simulink model "hdlcoder_ofdm_fft_eml"  (R2026a)
settings: Solver=FixedStepDiscrete  StopTime=5000
PreLoadFcn:
  | wordLength = 12;
  | fracLength = 6;
InitFcn:
  | TotalPoint= 512;
  | TotalStage= 9;
  | FFT_nt=numerictype(1,12, 6);
  | twiddle_Signed = 1;
  | twiddle_WordLength = 12;
  | twiddle_FractionLength = 10;
  | twiddle_nt=numerictype(1,12, 10);
undefined symbols (not defined in the file or in its folder): EbNodB, M, Tsym
libraries: hdlsllib x10, commdigbbndam3 x3, dspxfrm3 x2, commsink2 x2, commchan3 x1, simulink x1, commseqgen3 x1, dspindex x1, commrandsrc3 x1
(part 1 of 3)
Description:
  | OFDM Receiver with 512-Point Serial FFT
  | This model shows how to use Simulink(R) HDL Coder(TM) to check, generate,
  | and verify HDL code for a 512-point serial-FFT block built using the
  | MATLAB Function blocks and Simulink(R) blocks.
  | 
  | The 512-point serial-FFT block implements Radix-2 Dicimation-in-Time Cooley-Turkey algorithm.
  | It accepts streaming complex inputs and generate streaming complex outputs.
settings Model: FPTRunName=Active  Creator=The MathWorks, Inc.  LastModifiedBy=The MathWorks, Inc.
settings OptimizationCC: ConditionallyExecuteInputs=off  InitFltsAndDblsToZero=on  EfficientMapNaN2IntZero=off
settings DebuggingCC: AlgebraicLoopMsg=error  MultiTaskDSMMsg=warning  MultiTaskCondExecSysMsg=none  SingleTaskRateTransMsg=error  IntegerOverflowMsg=none  NonBusSignalsTreatedAsBus=error  IntegerSaturationMsg=none
settings HardwareCC: ProdHWDeviceType=32-bit Generic
settings GRTTargetCC: CombineOutputUpdateFcns=off  GRTInterface=on

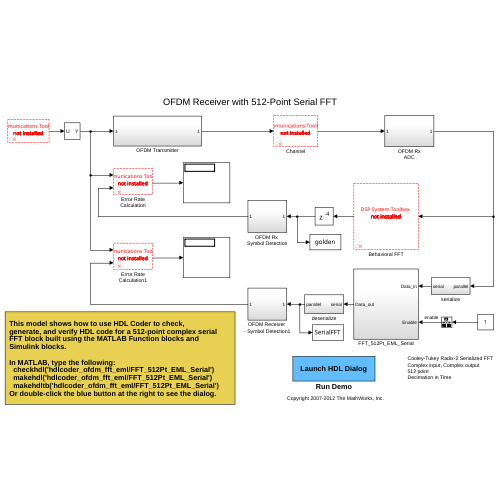
[thumbnail: Simulink's stored preview of the top-level diagram]
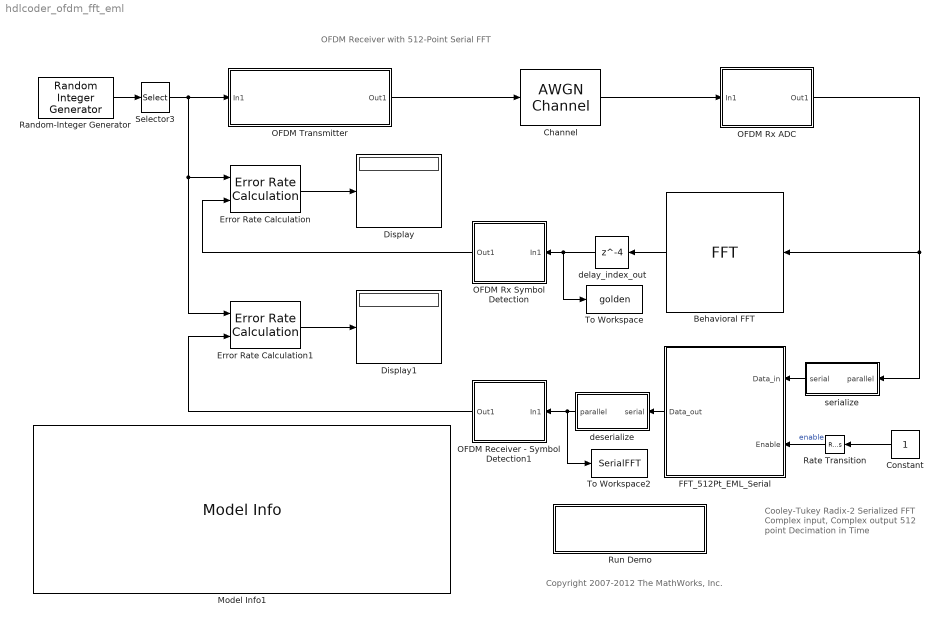
== system hdlcoder_ofdm_fft_eml ==
  note: OFDM Receiver with 512-Point Serial FFT
  note: Cooley-Tukey Radix-2 Serialized FFT
      | Complex input, Complex output
      | 512 point
      | Decimation in Time
  note: Copyright 2007-2012 The MathWorks, Inc.
  Behavioral FFT : dspxfrm3/FFT  FFTImplementation=Auto  CompMethod=Table lookup  TableOpt=NEW  TableOptActive=Speed  BitRevOrder=off  Normalize=off  InheritFFTLength=on  FFTLength=64  WrapInput=on  roundingMode=Floor  overflowMode=off  firstCoeffMode=Specify word length  firstCoeffWordLength=11  firstCoeffFracLength=10  firstCoeffDataTypeStr=fixdt(1,11)  firstCoeffLastDataTypeStr=fixdt(1,11)  prodOutputMode=Binary point scaling  prodOutputWordLength=24  prodOutputFracLength=16  prodOutputDataTypeStr=fixdt(1,24,16)  prodOutputLastDataTypeStr=fixdt(1,24,16)  accumMode=Binary point scaling  accumWordLength=25  accumFracLength=16  accumDataTypeStr=fixdt(1,25,16)  accumLastDataTypeStr=fixdt(1,25,16)  outputMode=Binary point scaling  outputWordLength=12  outputFracLength=6  outputDataTypeStr=fixdt(1,12,6)  outputMin=[]  outputMax=[]  outputLastDataTypeStr=fixdt(1,12,6)
  Channel : commchan3/AWGN Channel  LegacyMode=off  NoiseMethod="Signal to noise ratio  (SNR)"  noiseMode="Signal to noise ratio  (SNR)"  EbNo=10  EsNo=EbNodB+10*log10(log2(M))  SNR=10  BitsPerSymbol=1  SignalPower=1/512  SamplesPerSymbol=round(Tsym / 9.411765e-01)  SymbolPeriod=Tsym  VarianceSource=Parameter  Variance=10^(-0.1*15)/(2048*2)  RandomStream=mt19937ar with seed  Seed=54321  SimulateUsing=Code generation
  Constant : Constant  OutDataTypeStr=boolean  SampleTime=TotalPoint
  Display : Display
  Display1 : Display
  Error Rate Calculation : commsink2/Error Rate Calculation  N=384*4  st_delay=384  cp_mode=Entire frame  subframe=[]  PMode=Port  WsName=ErrorVec  RsMode2=off  stop=off  numErr=100  maxBits=1e6
  Error Rate Calculation1 : commsink2/Error Rate Calculation  N=384*4  st_delay=384  cp_mode=Entire frame  subframe=[]  PMode=Port  WsName=ErrorVec  RsMode2=off  stop=off  numErr=100  maxBits=1e6
  FFT_512Pt_EML_Serial : Subsystem
  Model Info1 : simulink/Model-Wide Utilities/Model Info  Frame=on  DisplayStringWithTags=|  HorizontalTextAlignment=Left  LeftAlignmentValue=0.02
      | This model shows how to use HDL Coder to check, 
      | generate, and verify HDL code for a 512-point complex serial
      | FFT block built using the MATLAB Function blocks and
      | Simulink blocks.
      | 
      | In MATLAB, type the following:
      |   checkhdl('hdlcoder_ofdm_fft_eml/FFT_512Pt_EML_Serial')
      |   makehdl('hdlcoder_ofdm_fft_eml/FFT_512Pt_EML_Serial')
      |   makehdltb('hdlcoder_ofdm_fft_eml/FFT_512Pt_EML_Serial')
      | Or double-click the blue button at the right to see the dialog.
  OFDM Receiver - Symbol Detection1 : Subsystem
  OFDM Rx ADC : Subsystem
  OFDM Rx Symbol Detection : Subsystem
  OFDM Transmitter : Subsystem
  Random-Integer Generator : commrandsrc3/Random Integer Generator  SetSize=64  SeedSource=Parameter  Seed=1234573  SampleTime=1  SamplesPerFrame=512  OutputDataType=uint8  SimulateUsing=Interpreted execution
  Rate Transition : RateTransition
  Run Demo : Subsystem
      settings: OpenFcn=hdldialog(bdroot)
      mask Display: disp('Launch HDL Dialog')
  Selector3 : Selector  InputPortWidth=512  IndexOptions=Index vector (dialog)  Indices=[1:384]  OutputSizes=1
  To Workspace : ToWorkspace  VariableName=golden  SampleTime=-1
      settings: MaxDataPoints=1
  To Workspace2 : ToWorkspace  VariableName=SerialFFT  SampleTime=-1
      settings: MaxDataPoints=1
  delay_index_out : Delay  DelayLength=4  SampleTime=512
  deserialize : Subsystem
  serialize : Subsystem
  wires:
  Channel/1 -> OFDM Rx ADC/1(In1)
  Random-Integer Generator/1 -> Selector3/1
  OFDM Transmitter/1(Out1) -> Channel/1
  Error Rate Calculation1/1 -> Display1/1
  Selector3/1 -> OFDM Transmitter/1(In1), Error Rate Calculation1/1, Error Rate Calculation/1
  FFT_512Pt_EML_Serial/1(Data_out) -> deserialize/1(serial)
  delay_index_out/1 -> OFDM Rx Symbol Detection/1(In1), To Workspace/1
  Behavioral FFT/1 -> delay_index_out/1
  Constant/1 -> Rate Transition/1
  Error Rate Calculation/1 -> Display/1
  serialize/1(serial) -> FFT_512Pt_EML_Serial/1(Data_in)
  Rate Transition/1 -> FFT_512Pt_EML_Serial/2(Enable)  "enable"
  OFDM Rx ADC/1(Out1) -> serialize/1(parallel), Behavioral FFT/1
  deserialize/1(parallel) -> OFDM Receiver - Symbol Detection1/1(In1), To Workspace2/1
  OFDM Rx Symbol Detection/1(Out1) -> Error Rate Calculation/2
  OFDM Receiver - Symbol Detection1/1(Out1) -> Error Rate Calculation1/2

== system hdlcoder_ofdm_fft_eml/FFT_512Pt_EML_Serial ==
  Data_in : Inport
  Enable : Inport  Port=2
  Serialized_FFT : Subsystem
  Terminator : Terminator
  Terminator1 : Terminator
  Data_out : Outport
  wires:
  Enable/1 -> Serialized_FFT/1(enable)
  Data_in/1 -> Serialized_FFT/2(data_in)  "serial_in"
  Serialized_FFT/1(data_en) -> Terminator/1
  Serialized_FFT/2(data_out) -> Data_out/1
  Serialized_FFT/3(Index_out) -> Terminator1/1

== system hdlcoder_ofdm_fft_eml/OFDM Receiver - Symbol Detection1 ==
  In1 : Inport
  Data Type Conversion4 : DataTypeConversion  OutDataTypeStr=uint8  SaturateOnIntegerOverflow=off  RndMeth=Floor
  Extract Data Carriers and Reorder1 : Selector  InputPortWidth=512  IndexOptions=Index vector (dialog)  Indices=[317:340 342:389 391:438 440:487 489:512 2:25 27:74 76:123 125:172 174:197]  OutputSizes=1
  Frame Conversion : FrameConversion
  RX Power Scaling1 : Gain  Gain=1/4
  Rectangular QAM Demodulator Baseband : commdigbbndam3/Rectangular QAM Demodulator Baseband  M=64  OutType=Integer  DecType=Hard decision  VarSource=Dialog  Variance=1  Dec=Gray  Mapping=[0:15]  PowType=Min. distance between symbols  MinDist=2  AvgPow=1  PeakPow=1  Ph=0  outDtype1=Inherit via internal rule  outDtype2=Inherit via internal rule  derotateFactorWordLen=16  derotateFactorDataTypeStr=Inherit: Same word length as input  derotateFactorLastDataTypeStr=Inherit: Same word length as input  denormFactorWordLen=16  denormFactorDataTypeStr=Inherit: Same word length as input  denormFactorLastDataTypeStr=Inherit: Same word length as input  prodOutWordLen=32  prodOutOverflowMode=Wrap  prodOutRoundingMode=Floor  prodOutOvFlMode=off  prodOutOvFlModeLastStrValue=off  sumWordLen=32
  Rx DAC : DataTypeConversion  OutDataTypeStr=double  SaturateOnIntegerOverflow=off  RndMeth=Floor
  Out1 : Outport
  wires:
  In1/1 -> Rx DAC/1
  Data Type Conversion4/1 -> Out1/1
  Extract Data Carriers and Reorder1/1 -> RX Power Scaling1/1
  RX Power Scaling1/1 -> Rectangular QAM Demodulator Baseband/1
  Frame Conversion/1 -> Extract Data Carriers and Reorder1/1
  Rx DAC/1 -> Frame Conversion/1
  Rectangular QAM Demodulator Baseband/1 -> Data Type Conversion4/1

== system hdlcoder_ofdm_fft_eml/OFDM Rx ADC ==
  In1 : Inport
  Frame Conversion1 : FrameConversion  OutFrame=Sample-based
  Remove Cyclic Prefix : Selector  NumberOfDimensions=2  InputPortWidth=80  IndexOptions=Index vector (dialog),Select all  Indices=[33:544],1  OutputSizes=1,1
  Rx ADC : DataTypeConversion  OutDataTypeStr=fixdt(1,wordLength,fracLength)  SaturateOnIntegerOverflow=off  RndMeth=Floor
  Out1 : Outport
  wires:
  Rx ADC/1 -> Frame Conversion1/1
  Frame Conversion1/1 -> Remove Cyclic Prefix/1
  Remove Cyclic Prefix/1 -> Out1/1
  In1/1 -> Rx ADC/1

== system hdlcoder_ofdm_fft_eml/OFDM Rx Symbol Detection ==
  In1 : Inport
  Data Type Conversion4 : DataTypeConversion  OutDataTypeStr=uint8  SaturateOnIntegerOverflow=off  RndMeth=Floor
  Extract Data Carriers and Reorder1 : Selector  InputPortWidth=512  IndexOptions=Index vector (dialog)  Indices=[317:340 342:389 391:438 440:487 489:512 2:25 27:74 76:123 125:172 174:197]  OutputSizes=1
  Frame Conversion : FrameConversion
  RX Power Scaling1 : Gain  Gain=1/4
  Rectangular QAM Demodulator Baseband : commdigbbndam3/Rectangular QAM Demodulator Baseband  M=64  OutType=Integer  DecType=Hard decision  VarSource=Dialog  Variance=1  Dec=Gray  Mapping=[0:15]  PowType=Min. distance between symbols  MinDist=2  AvgPow=1  PeakPow=1  Ph=0  outDtype1=Inherit via internal rule  outDtype2=Inherit via internal rule  derotateFactorWordLen=16  derotateFactorDataTypeStr=Inherit: Same word length as input  derotateFactorLastDataTypeStr=Inherit: Same word length as input  denormFactorWordLen=16  denormFactorDataTypeStr=Inherit: Same word length as input  denormFactorLastDataTypeStr=Inherit: Same word length as input  prodOutWordLen=32  prodOutOverflowMode=Wrap  prodOutRoundingMode=Floor  prodOutOvFlMode=off  prodOutOvFlModeLastStrValue=off  sumWordLen=32
  Rx DAC : DataTypeConversion  OutDataTypeStr=double  SaturateOnIntegerOverflow=off  RndMeth=Floor
  Out1 : Outport
  wires:
  Rectangular QAM Demodulator Baseband/1 -> Data Type Conversion4/1
  Rx DAC/1 -> Frame Conversion/1
  Frame Conversion/1 -> Extract Data Carriers and Reorder1/1
  RX Power Scaling1/1 -> Rectangular QAM Demodulator Baseband/1
  Extract Data Carriers and Reorder1/1 -> RX Power Scaling1/1
  Data Type Conversion4/1 -> Out1/1
  In1/1 -> Rx DAC/1

== system hdlcoder_ofdm_fft_eml/OFDM Transmitter ==
  In1 : Inport
  Append Cyclic Prefix : Selector  NumberOfDimensions=2  InputPortWidth=256  IndexOptions=Index vector (dialog),Select all  Indices=[481:512 1:512],1  OutputSizes=1,1
  IFFT : dspxfrm3/IFFT  FFTImplementation=Auto  CompMethod=Table lookup  TableOpt=HYBRID  TableOptActive=Speed  BitRevOrder=off  cs_in=off  Normalize=on  InheritFFTLength=on  FFTLength=64  WrapInput=on  mode=Complex  outSamplingMode=Frame based  roundingMode=Floor  overflowMode=off  firstCoeffMode=Specify word length  firstCoeffWordLength=16  firstCoeffFracLength=15  firstCoeffDataTypeStr=fixdt(1,16)  firstCoeffLastDataTypeStr=fixdt(1,16)  accumDataTypeStr=Inherit: Same as product output  accumLastDataTypeStr=Inherit: Same as product output  outputMin=[]  outputMax=[]
  Insert Pilots : Subsystem
  Rectangular QAM Modulator Baseband : commdigbbndam3/Rectangular QAM Modulator Baseband  M=64  InType=Integer  Enc=Gray  Mapping=[0:15]  PowType=Min. distance between symbols  MinDist=2  AvgPow=1  PeakPow=1  Ph=0  outDtype=double  outWordLen=16  outUDDataType=sfix(16)  outFracLenMode=Best precision  outFracLen=15  outDataTypeStr=double  outLastDataTypeStr=double
  TX Power Scaling : Gain  Gain=4
  Tx ADC : DataTypeConversion  OutDataTypeStr=fixdt(1,wordLength,fracLength)  SaturateOnIntegerOverflow=off  RndMeth=Floor
  Tx DAC : DataTypeConversion  OutDataTypeStr=double  SaturateOnIntegerOverflow=off  RndMeth=Floor
  Out1 : Outport
  wires:
  Rectangular QAM Modulator Baseband/1 -> Insert Pilots/1(In1)
  Insert Pilots/1(Out1) -> Tx ADC/1
  Tx ADC/1 -> IFFT/1
  TX Power Scaling/1 -> Append Cyclic Prefix/1
  IFFT/1 -> TX Power Scaling/1
  Append Cyclic Prefix/1 -> Tx DAC/1
  In1/1 -> Rectangular QAM Modulator Baseband/1
  Tx DAC/1 -> Out1/1

== system hdlcoder_ofdm_fft_eml/Run Demo ==

== system hdlcoder_ofdm_fft_eml/deserialize ==
  serial : Inport
  Buffer : Buffer  N=512  OutputFrames=off
  Frame Conversion : FrameConversion  OutFrame=Sample-based
  Rate Transition : RateTransition  Deterministic=off  OutPortSampleTime=TotalPoint
  delay_index_out : Delay  DelayLength=238
  tp0c9cbef0_20fa_4817_87de_7b2a1aa0b940 : FrameConversion
  parallel : Outport
  wires:
  delay_index_out/1 -> Buffer/1
  serial/1 -> delay_index_out/1
  Rate Transition/1 -> parallel/1
  Frame Conversion/1 -> Rate Transition/1
  Buffer/1 -> tp0c9cbef0_20fa_4817_87de_7b2a1aa0b940/1
  tp0c9cbef0_20fa_4817_87de_7b2a1aa0b940/1 -> Frame Conversion/1

== system hdlcoder_ofdm_fft_eml/serialize ==
  parallel : Inport
  Frame Conversion : FrameConversion
  Unbuffer : Unbuffer
  serial : Outport
  wires:
  parallel/1 -> Frame Conversion/1
  Frame Conversion/1 -> Unbuffer/1
  Unbuffer/1 -> serial/1

== system hdlcoder_ofdm_fft_eml/FFT_512Pt_EML_Serial/Serialized_FFT ==
  enable : Inport
  data_in : Inport  Port=2
  End_Stage_Reorder : Subsystem
  FFT_Stages : Subsystem
  Start_Stage_BitReverse : Subsystem
  data_en : Outport
  data_out : Outport  Port=2
  Index_out : Outport  Port=3
  wires:
  Start_Stage_BitReverse/1(data_en) -> FFT_Stages/1(enable)
  Start_Stage_BitReverse/2(data_out) -> FFT_Stages/2(data_in)
  enable/1 -> Start_Stage_BitReverse/1(enable)
  data_in/1 -> Start_Stage_BitReverse/2(data_in)
  FFT_Stages/1(data_en) -> End_Stage_Reorder/1(enable)
  FFT_Stages/2(data_out) -> End_Stage_Reorder/2(data_in)
  FFT_Stages/3(index_out) -> End_Stage_Reorder/3(data_in1)
  End_Stage_Reorder/1(data_en) -> data_en/1
  End_Stage_Reorder/2(data_out) -> data_out/1
  End_Stage_Reorder/3(index_out) -> Index_out/1

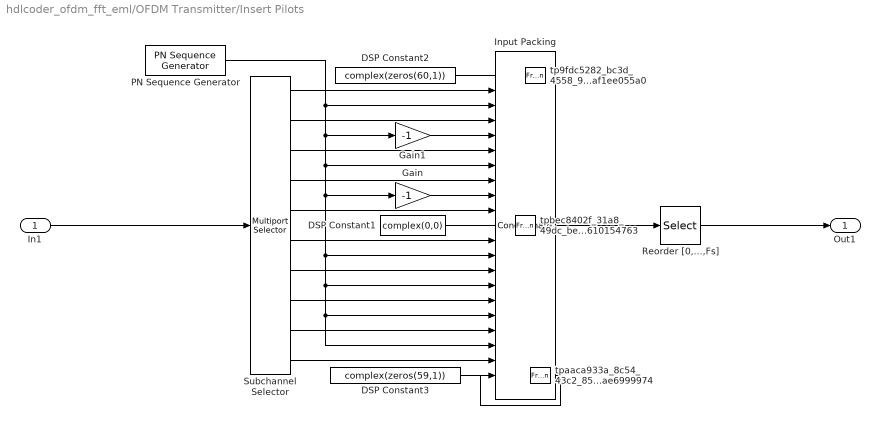
== system hdlcoder_ofdm_fft_eml/OFDM Transmitter/Insert Pilots ==
  In1 : Inport
  DSP Constant1 : Constant  Value=complex(0,0)  VectorParams1D=off
  DSP Constant2 : Constant  Value=complex(zeros(60,1))  VectorParams1D=off
  DSP Constant3 : Constant  Value=complex(zeros(59,1))  VectorParams1D=off
  Gain : Gain  Gain=-1
  Gain1 : Gain  Gain=-1
  Input Packing : Concatenate  NumInputs=21  Mode=Multidimensional array
  PN Sequence Generator : commseqgen3/PN Sequence Generator  poly=[1 0 0 0 0 0 0 0 0 0 0 0 0 1 1]  ini_sta=[1 0 0 1 0 1 0 1 0 0 0 0 0 0]  outBitMaskSource=Dialog parameter  shift=0  outVarSiz=off  maxOutSizeMode=Dialog parameter  maxOutSize=[10 1]  Ts=512  sampPerFrame=1  reset=off  bitPackedOutputs=off  outDataType=double  numPackedBits=8  bitPackDataSigned=off  bitPackedOutDType=double
  Reorder [0,...,Fs] : Selector  NumberOfDimensions=2  InputPortWidth=256  IndexOptions=Index vector (dialog),Select all  Indices=[257:512 1:256],1  OutputSizes=1,1
  Subchannel Selector : dspindex/Multiport Selector  rowsOrCols=Rows  idxCellArray={[1:24],[25:72],[73:120],[121:168],[169:192],[193:216],[217:264],[265:312],[313:360],[361:384]}  idxErrMode=Generate Error
  tp9fdc5282_bc3d_4558_90ac_c7af1ee055a0 : FrameConversion
  tpaaca933a_8c54_43c2_85ab_d0aae6999974 : FrameConversion
  tpbec8402f_31a8_49dc_be14_d26610154763 : FrameConversion
  Out1 : Outport
  wires:
  In1/1 -> Subchannel Selector/1
  PN Sequence Generator/1 -> Gain1/1, Gain/1, Input Packing/19, Input Packing/17, Input Packing/15, Input Packing/13, Input Packing/7, Input Packing/3
  Subchannel Selector/10 -> Input Packing/20
  Subchannel Selector/9 -> Input Packing/18
  Subchannel Selector/8 -> Input Packing/16
  Subchannel Selector/7 -> Input Packing/14
  Subchannel Selector/6 -> Input Packing/12
  Subchannel Selector/5 -> Input Packing/10
  Subchannel Selector/4 -> Input Packing/8
  Subchannel Selector/3 -> Input Packing/6
  Subchannel Selector/2 -> Input Packing/4
  Subchannel Selector/1 -> Input Packing/2
  Gain/1 -> Input Packing/9
  Gain1/1 -> Input Packing/5
  Input Packing/1 -> Reorder [0,...,Fs]/1
  Reorder [0,...,Fs]/1 -> Out1/1
  DSP Constant1/1 -> tpbec8402f_31a8_49dc_be14_d26610154763/1
  tpbec8402f_31a8_49dc_be14_d26610154763/1 -> Input Packing/11
  DSP Constant2/1 -> tp9fdc5282_bc3d_4558_90ac_c7af1ee055a0/1
  tp9fdc5282_bc3d_4558_90ac_c7af1ee055a0/1 -> Input Packing/1
  DSP Constant3/1 -> tpaaca933a_8c54_43c2_85ab_d0aae6999974/1
  tpaaca933a_8c54_43c2_85ab_d0aae6999974/1 -> Input Packing/21

== system hdlcoder_ofdm_fft_eml/FFT_512Pt_EML_Serial/Serialized_FFT/End_Stage_Reorder ==
  enable : Inport
  data_in : Inport  Port=2
  data_in1 : Inport  Port=3
  Data Type Conversion : DataTypeConversion  SaturateOnIntegerOverflow=off  RndMeth=Floor
  Data Type Conversion1 : DataTypeConversion  SaturateOnIntegerOverflow=off  RndMeth=Floor
  Dual Port RAM : hdlsllib/HDL RAMs/Simple Dual Port RAM  ram_size=TotalStage+1
  Reorder_Control_Logics : MATLAB Function  TreatAsAtomicUnit=on
  data_en : Outport
  data_out : Outport  Port=2
  index_out : Outport  Port=3
  wires:
  Data Type Conversion1/1 -> Dual Port RAM/4
  Data Type Conversion/1 -> Dual Port RAM/2
  Reorder_Control_Logics/4(mem_wr_din) -> Dual Port RAM/1
  data_in1/1 -> Reorder_Control_Logics/3(index_in)
  data_in/1 -> Reorder_Control_Logics/2(data_in)
  enable/1 -> Reorder_Control_Logics/1(enable)
  Reorder_Control_Logics/3(index_out) -> index_out/1
  Reorder_Control_Logics/2(data_out) -> data_out/1
  Reorder_Control_Logics/1(data_en) -> data_en/1
  Reorder_Control_Logics/7(mem_rd_addr) -> Data Type Conversion1/1
  Reorder_Control_Logics/6(mem_wr_en) -> Dual Port RAM/3
  Reorder_Control_Logics/5(mem_wr_addr) -> Data Type Conversion/1
  Dual Port RAM/1 -> Reorder_Control_Logics/4(mem_rd_dout)

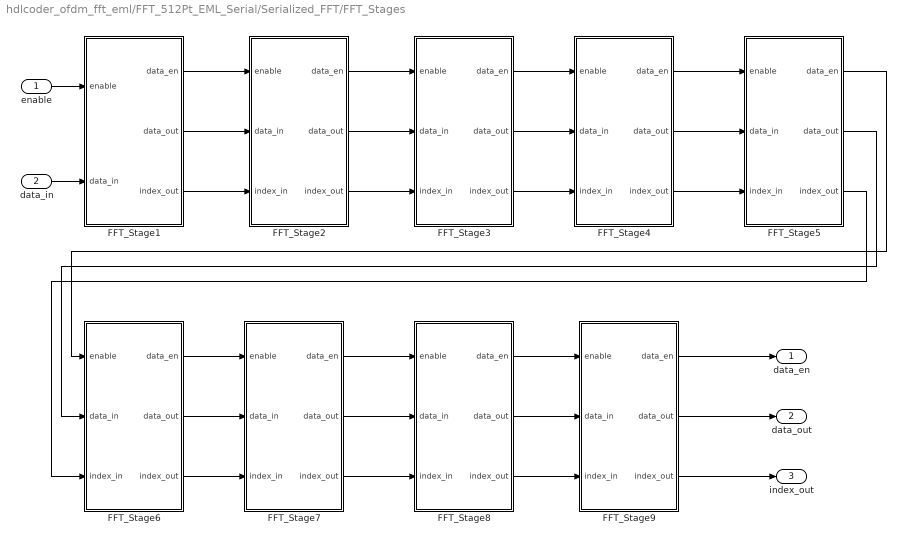
== system hdlcoder_ofdm_fft_eml/FFT_512Pt_EML_Serial/Serialized_FFT/FFT_Stages ==
  enable : Inport
  data_in : Inport  Port=2
  FFT_Stage1 : Subsystem
  FFT_Stage2 : Subsystem
  FFT_Stage3 : Subsystem
  FFT_Stage4 : Subsystem
  FFT_Stage5 : Subsystem
  FFT_Stage6 : Subsystem
  FFT_Stage7 : Subsystem
  FFT_Stage8 : Subsystem
  FFT_Stage9 : Subsystem
  data_en : Outport
  data_out : Outport  Port=2
  index_out : Outport  Port=3
  wires:
  enable/1 -> FFT_Stage1/1(enable)
  data_in/1 -> FFT_Stage1/2(data_in)
  FFT_Stage1/1(data_en) -> FFT_Stage2/1(enable)
  FFT_Stage1/2(data_out) -> FFT_Stage2/2(data_in)
  FFT_Stage1/3(index_out) -> FFT_Stage2/3(index_in)
  FFT_Stage2/1(data_en) -> FFT_Stage3/1(enable)
  FFT_Stage2/2(data_out) -> FFT_Stage3/2(data_in)
  FFT_Stage2/3(index_out) -> FFT_Stage3/3(index_in)
  FFT_Stage3/1(data_en) -> FFT_Stage4/1(enable)
  FFT_Stage3/2(data_out) -> FFT_Stage4/2(data_in)
  FFT_Stage3/3(index_out) -> FFT_Stage4/3(index_in)
  FFT_Stage4/1(data_en) -> FFT_Stage5/1(enable)
  FFT_Stage4/2(data_out) -> FFT_Stage5/2(data_in)
  FFT_Stage4/3(index_out) -> FFT_Stage5/3(index_in)
  FFT_Stage6/1(data_en) -> FFT_Stage7/1(enable)
  FFT_Stage6/2(data_out) -> FFT_Stage7/2(data_in)
  FFT_Stage6/3(index_out) -> FFT_Stage7/3(index_in)
  FFT_Stage7/1(data_en) -> FFT_Stage8/1(enable)
  FFT_Stage7/2(data_out) -> FFT_Stage8/2(data_in)
  FFT_Stage7/3(index_out) -> FFT_Stage8/3(index_in)
  FFT_Stage8/1(data_en) -> FFT_Stage9/1(enable)
  FFT_Stage8/2(data_out) -> FFT_Stage9/2(data_in)
  FFT_Stage8/3(index_out) -> FFT_Stage9/3(index_in)
  FFT_Stage5/1(data_en) -> FFT_Stage6/1(enable)
  FFT_Stage5/2(data_out) -> FFT_Stage6/2(data_in)
  FFT_Stage5/3(index_out) -> FFT_Stage6/3(index_in)
  FFT_Stage9/1(data_en) -> data_en/1
  FFT_Stage9/2(data_out) -> data_out/1
  FFT_Stage9/3(index_out) -> index_out/1

== system hdlcoder_ofdm_fft_eml/FFT_512Pt_EML_Serial/Serialized_FFT/Start_Stage_BitReverse ==
  enable : Inport
  data_in : Inport  Port=2
  BitReverse_Control_Logics : MATLAB Function  TreatAsAtomicUnit=on
  Dual Port RAM : hdlsllib/HDL RAMs/Simple Dual Port RAM  ram_size=TotalStage+1
  delay_data_en : UnitDelay
  delay_data_out : UnitDelay
  data_en : Outport
  data_out : Outport  Port=2
  wires:
  BitReverse_Control_Logics/1(data_en) -> delay_data_en/1
  BitReverse_Control_Logics/2(data_out) -> delay_data_out/1
  enable/1 -> BitReverse_Control_Logics/1(enable)
  data_in/1 -> BitReverse_Control_Logics/2(data_in)
  BitReverse_Control_Logics/3(mem_wr_din) -> Dual Port RAM/1
  BitReverse_Control_Logics/6(mem_rd_addr) -> Dual Port RAM/4
  BitReverse_Control_Logics/5(mem_wr_en) -> Dual Port RAM/3
  BitReverse_Control_Logics/4(mem_wr_addr) -> Dual Port RAM/2
  delay_data_en/1 -> data_en/1
  delay_data_out/1 -> data_out/1
  Dual Port RAM/1 -> BitReverse_Control_Logics/3(mem_rd_dout)

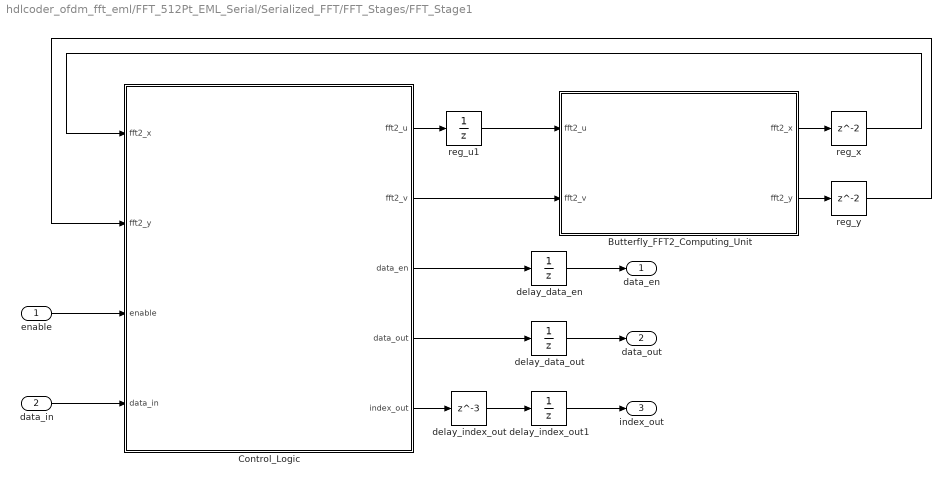
== system hdlcoder_ofdm_fft_eml/FFT_512Pt_EML_Serial/Serialized_FFT/FFT_Stages/FFT_Stage1 ==
  enable : Inport
  data_in : Inport  Port=2
  Butterfly_FFT2_Computing_Unit : MATLAB Function  TreatAsAtomicUnit=on
  Control_Logic : MATLAB Function  TreatAsAtomicUnit=on
  delay_data_en : UnitDelay
  delay_data_out : UnitDelay
  delay_index_out : Delay  DelayLength=3
  delay_index_out1 : UnitDelay
  reg_u1 : UnitDelay
  reg_x : Delay
  reg_y : Delay
  data_en : Outport
  data_out : Outport  Port=2
  index_out : Outport  Port=3
  wires:
  Butterfly_FFT2_Computing_Unit/1(fft2_x) -> reg_x/1
  Butterfly_FFT2_Computing_Unit/2(fft2_y) -> reg_y/1
  delay_index_out/1 -> delay_index_out1/1
  reg_x/1 -> Control_Logic/1(fft2_x)
  reg_y/1 -> Control_Logic/2(fft2_y)
  delay_data_en/1 -> data_en/1
  delay_data_out/1 -> data_out/1
  delay_index_out1/1 -> index_out/1
  Control_Logic/1(fft2_u) -> reg_u1/1
  Control_Logic/2(fft2_v) -> Butterfly_FFT2_Computing_Unit/2(fft2_v)
  reg_u1/1 -> Butterfly_FFT2_Computing_Unit/1(fft2_u)
  enable/1 -> Control_Logic/3(enable)
  data_in/1 -> Control_Logic/4(data_in)
  Control_Logic/3(data_en) -> delay_data_en/1
  Control_Logic/4(data_out) -> delay_data_out/1
  Control_Logic/5(index_out) -> delay_index_out/1

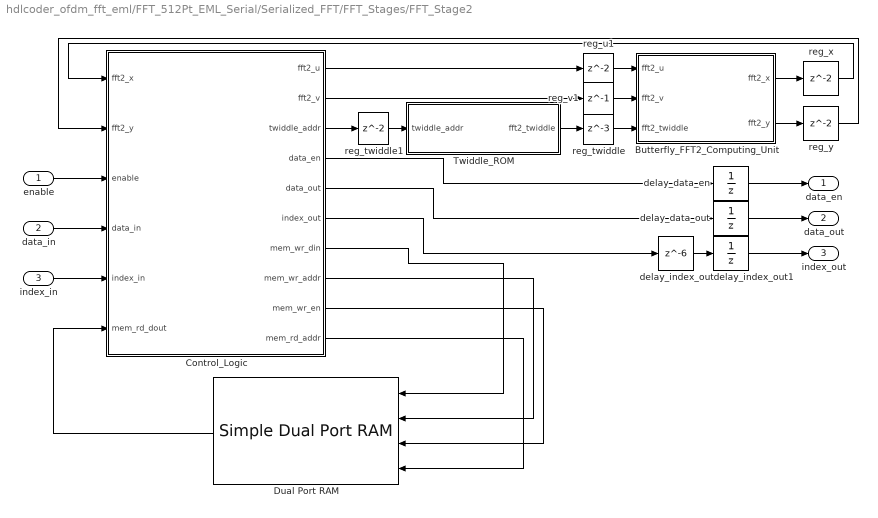
== system hdlcoder_ofdm_fft_eml/FFT_512Pt_EML_Serial/Serialized_FFT/FFT_Stages/FFT_Stage2 ==
  enable : Inport
  data_in : Inport  Port=2
  index_in : Inport  Port=3
  Butterfly_FFT2_Computing_Unit : MATLAB Function  TreatAsAtomicUnit=on
  Control_Logic : MATLAB Function  TreatAsAtomicUnit=on
  Dual Port RAM : hdlsllib/HDL RAMs/Simple Dual Port RAM  ram_size=2
  Twiddle_ROM : MATLAB Function  TreatAsAtomicUnit=on
  delay_data_en : UnitDelay
  delay_data_out : UnitDelay
  delay_index_out : Delay  DelayLength=6
  delay_index_out1 : UnitDelay
  reg_twiddle : Delay  DelayLength=3
  reg_twiddle1 : Delay
  reg_u1 : Delay
  reg_v1 : Delay  DelayLength=1
  reg_x : Delay
  reg_y : Delay
  data_en : Outport
  data_out : Outport  Port=2
  index_out : Outport  Port=3
  wires:
  Control_Logic/7(mem_wr_din) -> Dual Port RAM/1
  Control_Logic/6(index_out) -> delay_index_out/1
  Control_Logic/5(data_out) -> delay_data_out/1
  Control_Logic/4(data_en) -> delay_data_en/1
  Control_Logic/2(fft2_v) -> reg_v1/1
  reg_v1/1 -> Butterfly_FFT2_Computing_Unit/2(fft2_v)
  Dual Port RAM/1 -> Control_Logic/6(mem_rd_dout)
  reg_twiddle1/1 -> Twiddle_ROM/1(twiddle_addr)
  Twiddle_ROM/1(fft2_twiddle) -> reg_twiddle/1
  delay_index_out1/1 -> index_out/1
  delay_data_out/1 -> data_out/1
  delay_data_en/1 -> data_en/1
  index_in/1 -> Control_Logic/5(index_in)
  data_in/1 -> Control_Logic/4(data_in)
  enable/1 -> Control_Logic/3(enable)
  reg_y/1 -> Control_Logic/2(fft2_y)
  reg_x/1 -> Control_Logic/1(fft2_x)
  reg_twiddle/1 -> Butterfly_FFT2_Computing_Unit/3(fft2_twiddle)
  Control_Logic/3(twiddle_addr) -> reg_twiddle1/1
  reg_u1/1 -> Butterfly_FFT2_Computing_Unit/1(fft2_u)
  delay_index_out/1 -> delay_index_out1/1
  Butterfly_FFT2_Computing_Unit/2(fft2_y) -> reg_y/1
  Butterfly_FFT2_Computing_Unit/1(fft2_x) -> reg_x/1
  Control_Logic/1(fft2_u) -> reg_u1/1
  Control_Logic/10(mem_rd_addr) -> Dual Port RAM/4
  Control_Logic/9(mem_wr_en) -> Dual Port RAM/3
  Control_Logic/8(mem_wr_addr) -> Dual Port RAM/2

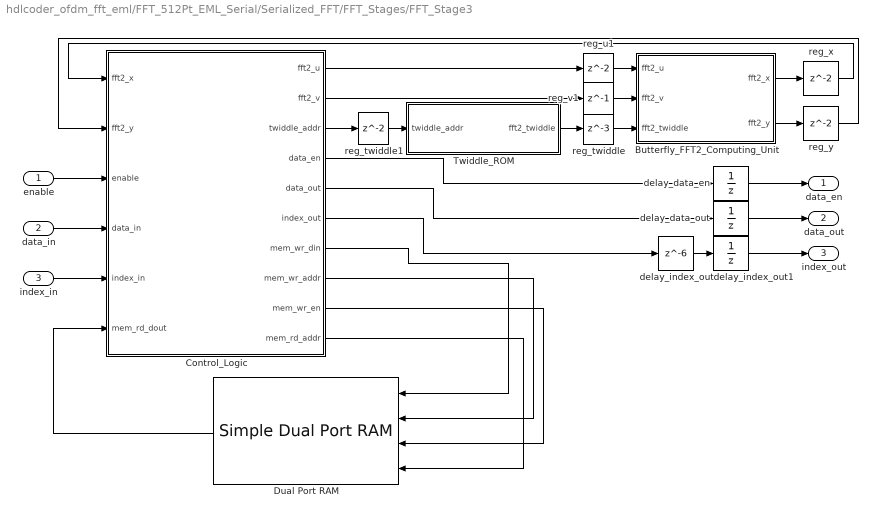
== system hdlcoder_ofdm_fft_eml/FFT_512Pt_EML_Serial/Serialized_FFT/FFT_Stages/FFT_Stage3 ==
  enable : Inport
  data_in : Inport  Port=2
  index_in : Inport  Port=3
  Butterfly_FFT2_Computing_Unit : MATLAB Function  TreatAsAtomicUnit=on
  Control_Logic : MATLAB Function  TreatAsAtomicUnit=on
  Dual Port RAM : hdlsllib/HDL RAMs/Simple Dual Port RAM  ram_size=3
  Twiddle_ROM : MATLAB Function  TreatAsAtomicUnit=on
  delay_data_en : UnitDelay
  delay_data_out : UnitDelay
  delay_index_out : Delay  DelayLength=6
  delay_index_out1 : UnitDelay
  reg_twiddle : Delay  DelayLength=3
  reg_twiddle1 : Delay
  reg_u1 : Delay
  reg_v1 : Delay  DelayLength=1
  reg_x : Delay
  reg_y : Delay
  data_en : Outport
  data_out : Outport  Port=2
  index_out : Outport  Port=3
  wires:
  Control_Logic/8(mem_wr_addr) -> Dual Port RAM/2
  Control_Logic/9(mem_wr_en) -> Dual Port RAM/3
  Control_Logic/10(mem_rd_addr) -> Dual Port RAM/4
  Control_Logic/1(fft2_u) -> reg_u1/1
  Butterfly_FFT2_Computing_Unit/1(fft2_x) -> reg_x/1
  Butterfly_FFT2_Computing_Unit/2(fft2_y) -> reg_y/1
  delay_index_out/1 -> delay_index_out1/1
  reg_u1/1 -> Butterfly_FFT2_Computing_Unit/1(fft2_u)
  Control_Logic/3(twiddle_addr) -> reg_twiddle1/1
  reg_twiddle/1 -> Butterfly_FFT2_Computing_Unit/3(fft2_twiddle)
  reg_x/1 -> Control_Logic/1(fft2_x)
  reg_y/1 -> Control_Logic/2(fft2_y)
  enable/1 -> Control_Logic/3(enable)
  data_in/1 -> Control_Logic/4(data_in)
  index_in/1 -> Control_Logic/5(index_in)
  delay_data_en/1 -> data_en/1
  delay_data_out/1 -> data_out/1
  delay_index_out1/1 -> index_out/1
  Twiddle_ROM/1(fft2_twiddle) -> reg_twiddle/1
  reg_twiddle1/1 -> Twiddle_ROM/1(twiddle_addr)
  Dual Port RAM/1 -> Control_Logic/6(mem_rd_dout)
  reg_v1/1 -> Butterfly_FFT2_Computing_Unit/2(fft2_v)
  Control_Logic/2(fft2_v) -> reg_v1/1
  Control_Logic/4(data_en) -> delay_data_en/1
  Control_Logic/5(data_out) -> delay_data_out/1
  Control_Logic/6(index_out) -> delay_index_out/1
  Control_Logic/7(mem_wr_din) -> Dual Port RAM/1

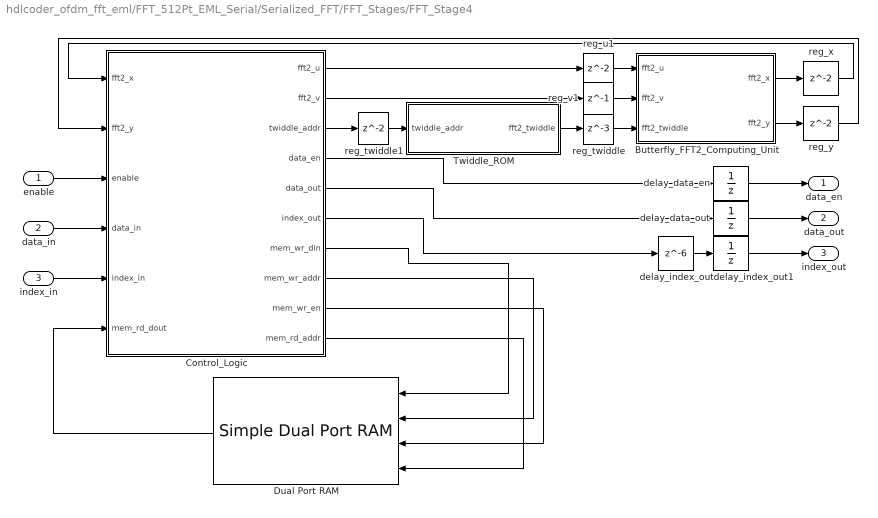
== system hdlcoder_ofdm_fft_eml/FFT_512Pt_EML_Serial/Serialized_FFT/FFT_Stages/FFT_Stage4 ==
  enable : Inport
  data_in : Inport  Port=2
  index_in : Inport  Port=3
  Butterfly_FFT2_Computing_Unit : MATLAB Function  TreatAsAtomicUnit=on
  Control_Logic : MATLAB Function  TreatAsAtomicUnit=on
  Dual Port RAM : hdlsllib/HDL RAMs/Simple Dual Port RAM  ram_size=4
  Twiddle_ROM : MATLAB Function  TreatAsAtomicUnit=on
  delay_data_en : UnitDelay
  delay_data_out : UnitDelay
  delay_index_out : Delay  DelayLength=6
  delay_index_out1 : UnitDelay
  reg_twiddle : Delay  DelayLength=3
  reg_twiddle1 : Delay
  reg_u1 : Delay
  reg_v1 : Delay  DelayLength=1
  reg_x : Delay
  reg_y : Delay
  data_en : Outport
  data_out : Outport  Port=2
  index_out : Outport  Port=3
  wires:
  Control_Logic/7(mem_wr_din) -> Dual Port RAM/1
  Control_Logic/6(index_out) -> delay_index_out/1
  Control_Logic/5(data_out) -> delay_data_out/1
  Control_Logic/4(data_en) -> delay_data_en/1
  Control_Logic/2(fft2_v) -> reg_v1/1
  reg_v1/1 -> Butterfly_FFT2_Computing_Unit/2(fft2_v)
  Dual Port RAM/1 -> Control_Logic/6(mem_rd_dout)
  reg_twiddle1/1 -> Twiddle_ROM/1(twiddle_addr)
  Twiddle_ROM/1(fft2_twiddle) -> reg_twiddle/1
  delay_index_out1/1 -> index_out/1
  delay_data_out/1 -> data_out/1
  delay_data_en/1 -> data_en/1
  index_in/1 -> Control_Logic/5(index_in)
  data_in/1 -> Control_Logic/4(data_in)
  enable/1 -> Control_Logic/3(enable)
  reg_y/1 -> Control_Logic/2(fft2_y)
  reg_x/1 -> Control_Logic/1(fft2_x)
  reg_twiddle/1 -> Butterfly_FFT2_Computing_Unit/3(fft2_twiddle)
  Control_Logic/3(twiddle_addr) -> reg_twiddle1/1
  reg_u1/1 -> Butterfly_FFT2_Computing_Unit/1(fft2_u)
  delay_index_out/1 -> delay_index_out1/1
  Butterfly_FFT2_Computing_Unit/2(fft2_y) -> reg_y/1
  Butterfly_FFT2_Computing_Unit/1(fft2_x) -> reg_x/1
  Control_Logic/1(fft2_u) -> reg_u1/1
  Control_Logic/10(mem_rd_addr) -> Dual Port RAM/4
  Control_Logic/9(mem_wr_en) -> Dual Port RAM/3
  Control_Logic/8(mem_wr_addr) -> Dual Port RAM/2

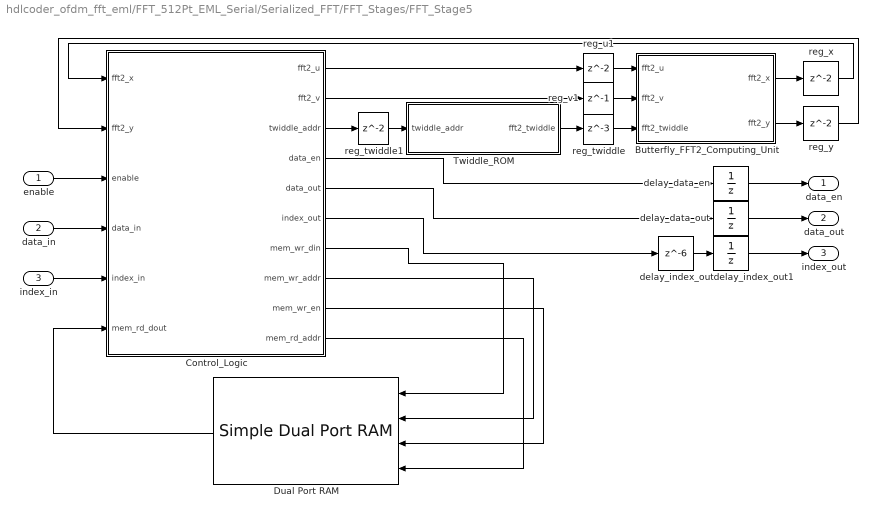
== system hdlcoder_ofdm_fft_eml/FFT_512Pt_EML_Serial/Serialized_FFT/FFT_Stages/FFT_Stage5 ==
  enable : Inport
  data_in : Inport  Port=2
  index_in : Inport  Port=3
  Butterfly_FFT2_Computing_Unit : MATLAB Function  TreatAsAtomicUnit=on
  Control_Logic : MATLAB Function  TreatAsAtomicUnit=on
  Dual Port RAM : hdlsllib/HDL RAMs/Simple Dual Port RAM  ram_size=5
  Twiddle_ROM : MATLAB Function  TreatAsAtomicUnit=on
  delay_data_en : UnitDelay
  delay_data_out : UnitDelay
  delay_index_out : Delay  DelayLength=6
  delay_index_out1 : UnitDelay
  reg_twiddle : Delay  DelayLength=3
  reg_twiddle1 : Delay
  reg_u1 : Delay
  reg_v1 : Delay  DelayLength=1
  reg_x : Delay
  reg_y : Delay
  data_en : Outport
  data_out : Outport  Port=2
  index_out : Outport  Port=3
  wires:
  Control_Logic/8(mem_wr_addr) -> Dual Port RAM/2
  Control_Logic/9(mem_wr_en) -> Dual Port RAM/3
  Control_Logic/10(mem_rd_addr) -> Dual Port RAM/4
  Control_Logic/1(fft2_u) -> reg_u1/1
  Butterfly_FFT2_Computing_Unit/1(fft2_x) -> reg_x/1
  Butterfly_FFT2_Computing_Unit/2(fft2_y) -> reg_y/1
  delay_index_out/1 -> delay_index_out1/1
  reg_u1/1 -> Butterfly_FFT2_Computing_Unit/1(fft2_u)
  Control_Logic/3(twiddle_addr) -> reg_twiddle1/1
  reg_twiddle/1 -> Butterfly_FFT2_Computing_Unit/3(fft2_twiddle)
  reg_x/1 -> Control_Logic/1(fft2_x)
  reg_y/1 -> Control_Logic/2(fft2_y)
  enable/1 -> Control_Logic/3(enable)
  data_in/1 -> Control_Logic/4(data_in)
  index_in/1 -> Control_Logic/5(index_in)
  delay_data_en/1 -> data_en/1
  delay_data_out/1 -> data_out/1
  delay_index_out1/1 -> index_out/1
  Twiddle_ROM/1(fft2_twiddle) -> reg_twiddle/1
  reg_twiddle1/1 -> Twiddle_ROM/1(twiddle_addr)
  Dual Port RAM/1 -> Control_Logic/6(mem_rd_dout)
  reg_v1/1 -> Butterfly_FFT2_Computing_Unit/2(fft2_v)
  Control_Logic/2(fft2_v) -> reg_v1/1
  Control_Logic/4(data_en) -> delay_data_en/1
  Control_Logic/5(data_out) -> delay_data_out/1
  Control_Logic/6(index_out) -> delay_index_out/1
  Control_Logic/7(mem_wr_din) -> Dual Port RAM/1

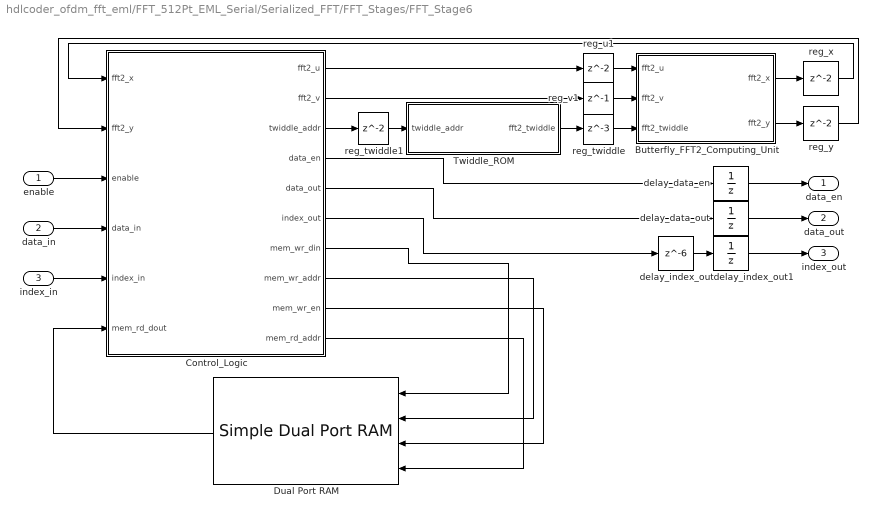
== system hdlcoder_ofdm_fft_eml/FFT_512Pt_EML_Serial/Serialized_FFT/FFT_Stages/FFT_Stage6 ==
  enable : Inport
  data_in : Inport  Port=2
  index_in : Inport  Port=3
  Butterfly_FFT2_Computing_Unit : MATLAB Function  TreatAsAtomicUnit=on
  Control_Logic : MATLAB Function  TreatAsAtomicUnit=on
  Dual Port RAM : hdlsllib/HDL RAMs/Simple Dual Port RAM  ram_size=6
  Twiddle_ROM : MATLAB Function  TreatAsAtomicUnit=on
  delay_data_en : UnitDelay
  delay_data_out : UnitDelay
  delay_index_out : Delay  DelayLength=6
  delay_index_out1 : UnitDelay
  reg_twiddle : Delay  DelayLength=3
  reg_twiddle1 : Delay
  reg_u1 : Delay
  reg_v1 : Delay  DelayLength=1
  reg_x : Delay
  reg_y : Delay
  data_en : Outport
  data_out : Outport  Port=2
  index_out : Outport  Port=3
  wires:
  Control_Logic/7(mem_wr_din) -> Dual Port RAM/1
  Control_Logic/6(index_out) -> delay_index_out/1
  Control_Logic/5(data_out) -> delay_data_out/1
  Control_Logic/4(data_en) -> delay_data_en/1
  Control_Logic/2(fft2_v) -> reg_v1/1
  reg_v1/1 -> Butterfly_FFT2_Computing_Unit/2(fft2_v)
  Dual Port RAM/1 -> Control_Logic/6(mem_rd_dout)
  reg_twiddle1/1 -> Twiddle_ROM/1(twiddle_addr)
  Twiddle_ROM/1(fft2_twiddle) -> reg_twiddle/1
  delay_index_out1/1 -> index_out/1
  delay_data_out/1 -> data_out/1
  delay_data_en/1 -> data_en/1
  index_in/1 -> Control_Logic/5(index_in)
  data_in/1 -> Control_Logic/4(data_in)
  enable/1 -> Control_Logic/3(enable)
  reg_y/1 -> Control_Logic/2(fft2_y)
  reg_x/1 -> Control_Logic/1(fft2_x)
  reg_twiddle/1 -> Butterfly_FFT2_Computing_Unit/3(fft2_twiddle)
  Control_Logic/3(twiddle_addr) -> reg_twiddle1/1
  reg_u1/1 -> Butterfly_FFT2_Computing_Unit/1(fft2_u)
  delay_index_out/1 -> delay_index_out1/1
  Butterfly_FFT2_Computing_Unit/2(fft2_y) -> reg_y/1
  Butterfly_FFT2_Computing_Unit/1(fft2_x) -> reg_x/1
  Control_Logic/1(fft2_u) -> reg_u1/1
  Control_Logic/10(mem_rd_addr) -> Dual Port RAM/4
  Control_Logic/9(mem_wr_en) -> Dual Port RAM/3
  Control_Logic/8(mem_wr_addr) -> Dual Port RAM/2

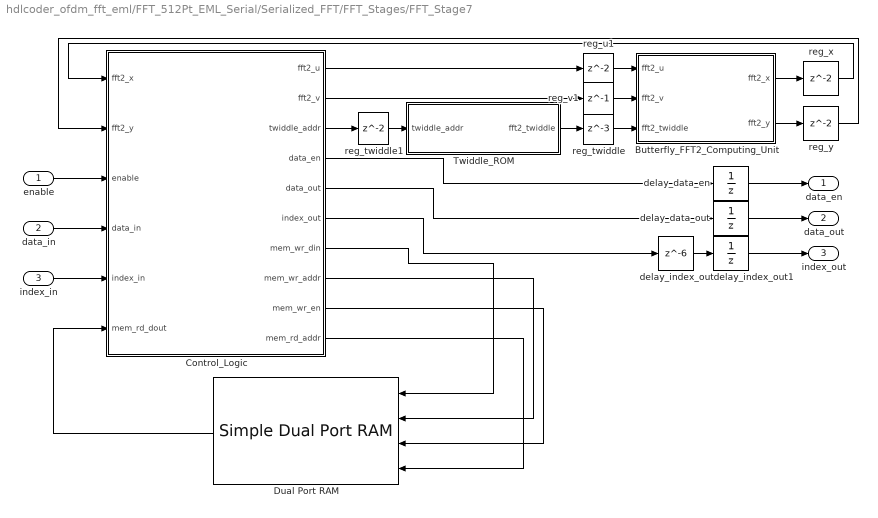
== system hdlcoder_ofdm_fft_eml/FFT_512Pt_EML_Serial/Serialized_FFT/FFT_Stages/FFT_Stage7 ==
  enable : Inport
  data_in : Inport  Port=2
  index_in : Inport  Port=3
  Butterfly_FFT2_Computing_Unit : MATLAB Function  TreatAsAtomicUnit=on
  Control_Logic : MATLAB Function  TreatAsAtomicUnit=on
  Dual Port RAM : hdlsllib/HDL RAMs/Simple Dual Port RAM  ram_size=7
  Twiddle_ROM : MATLAB Function  TreatAsAtomicUnit=on
  delay_data_en : UnitDelay
  delay_data_out : UnitDelay
  delay_index_out : Delay  DelayLength=6
  delay_index_out1 : UnitDelay
  reg_twiddle : Delay  DelayLength=3
  reg_twiddle1 : Delay
  reg_u1 : Delay
  reg_v1 : Delay  DelayLength=1
  reg_x : Delay
  reg_y : Delay
  data_en : Outport
  data_out : Outport  Port=2
  index_out : Outport  Port=3
  wires:
  Control_Logic/8(mem_wr_addr) -> Dual Port RAM/2
  Control_Logic/9(mem_wr_en) -> Dual Port RAM/3
  Control_Logic/10(mem_rd_addr) -> Dual Port RAM/4
  Control_Logic/1(fft2_u) -> reg_u1/1
  Butterfly_FFT2_Computing_Unit/1(fft2_x) -> reg_x/1
  Butterfly_FFT2_Computing_Unit/2(fft2_y) -> reg_y/1
  delay_index_out/1 -> delay_index_out1/1
  reg_u1/1 -> Butterfly_FFT2_Computing_Unit/1(fft2_u)
  Control_Logic/3(twiddle_addr) -> reg_twiddle1/1
  reg_twiddle/1 -> Butterfly_FFT2_Computing_Unit/3(fft2_twiddle)
  reg_x/1 -> Control_Logic/1(fft2_x)
  reg_y/1 -> Control_Logic/2(fft2_y)
  enable/1 -> Control_Logic/3(enable)
  data_in/1 -> Control_Logic/4(data_in)
  index_in/1 -> Control_Logic/5(index_in)
  delay_data_en/1 -> data_en/1
  delay_data_out/1 -> data_out/1
  delay_index_out1/1 -> index_out/1
  Twiddle_ROM/1(fft2_twiddle) -> reg_twiddle/1
  reg_twiddle1/1 -> Twiddle_ROM/1(twiddle_addr)
  Dual Port RAM/1 -> Control_Logic/6(mem_rd_dout)
  reg_v1/1 -> Butterfly_FFT2_Computing_Unit/2(fft2_v)
  Control_Logic/2(fft2_v) -> reg_v1/1
  Control_Logic/4(data_en) -> delay_data_en/1
  Control_Logic/5(data_out) -> delay_data_out/1
  Control_Logic/6(index_out) -> delay_index_out/1
  Control_Logic/7(mem_wr_din) -> Dual Port RAM/1

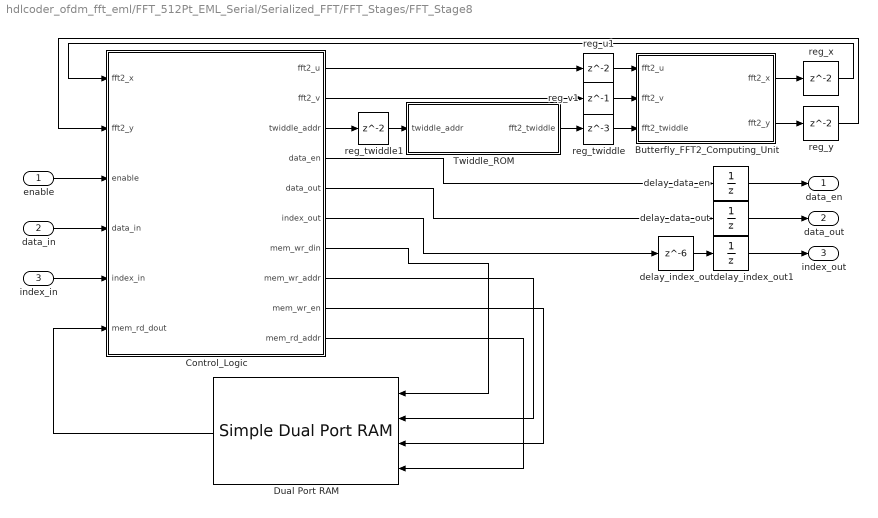
== system hdlcoder_ofdm_fft_eml/FFT_512Pt_EML_Serial/Serialized_FFT/FFT_Stages/FFT_Stage8 ==
  enable : Inport
  data_in : Inport  Port=2
  index_in : Inport  Port=3
  Butterfly_FFT2_Computing_Unit : MATLAB Function  TreatAsAtomicUnit=on
  Control_Logic : MATLAB Function  TreatAsAtomicUnit=on
  Dual Port RAM : hdlsllib/HDL RAMs/Simple Dual Port RAM  ram_size=8
  Twiddle_ROM : MATLAB Function  TreatAsAtomicUnit=on
  delay_data_en : UnitDelay
  delay_data_out : UnitDelay
  delay_index_out : Delay  DelayLength=6
  delay_index_out1 : UnitDelay
  reg_twiddle : Delay  DelayLength=3
  reg_twiddle1 : Delay
  reg_u1 : Delay
  reg_v1 : Delay  DelayLength=1
  reg_x : Delay
  reg_y : Delay
  data_en : Outport
  data_out : Outport  Port=2
  index_out : Outport  Port=3
  wires:
  Control_Logic/7(mem_wr_din) -> Dual Port RAM/1
  Control_Logic/6(index_out) -> delay_index_out/1
  Control_Logic/5(data_out) -> delay_data_out/1
  Control_Logic/4(data_en) -> delay_data_en/1
  Control_Logic/2(fft2_v) -> reg_v1/1
  reg_v1/1 -> Butterfly_FFT2_Computing_Unit/2(fft2_v)
  Dual Port RAM/1 -> Control_Logic/6(mem_rd_dout)
  reg_twiddle1/1 -> Twiddle_ROM/1(twiddle_addr)
  Twiddle_ROM/1(fft2_twiddle) -> reg_twiddle/1
  delay_index_out1/1 -> index_out/1
  delay_data_out/1 -> data_out/1
  delay_data_en/1 -> data_en/1
  index_in/1 -> Control_Logic/5(index_in)
  data_in/1 -> Control_Logic/4(data_in)
  enable/1 -> Control_Logic/3(enable)
  reg_y/1 -> Control_Logic/2(fft2_y)
  reg_x/1 -> Control_Logic/1(fft2_x)
  reg_twiddle/1 -> Butterfly_FFT2_Computing_Unit/3(fft2_twiddle)
  Control_Logic/3(twiddle_addr) -> reg_twiddle1/1
  reg_u1/1 -> Butterfly_FFT2_Computing_Unit/1(fft2_u)
  delay_index_out/1 -> delay_index_out1/1
  Butterfly_FFT2_Computing_Unit/2(fft2_y) -> reg_y/1
  Butterfly_FFT2_Computing_Unit/1(fft2_x) -> reg_x/1
  Control_Logic/1(fft2_u) -> reg_u1/1
  Control_Logic/10(mem_rd_addr) -> Dual Port RAM/4
  Control_Logic/9(mem_wr_en) -> Dual Port RAM/3
  Control_Logic/8(mem_wr_addr) -> Dual Port RAM/2

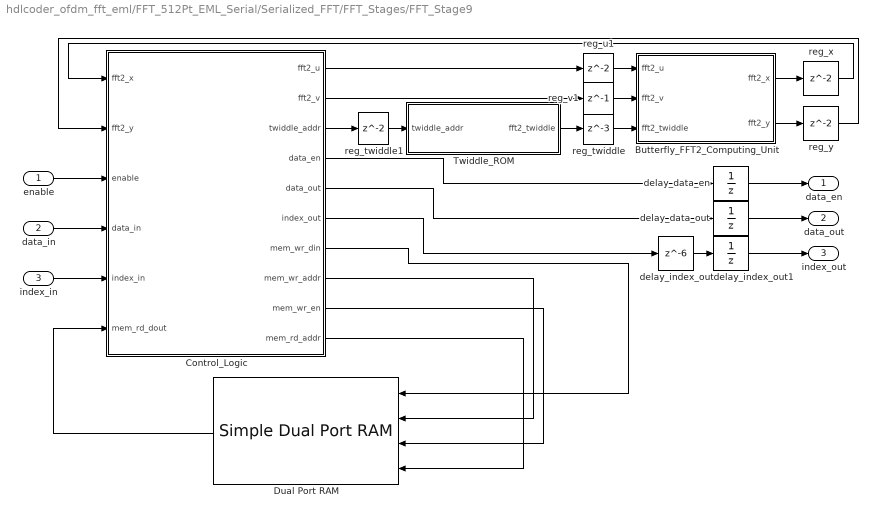
== system hdlcoder_ofdm_fft_eml/FFT_512Pt_EML_Serial/Serialized_FFT/FFT_Stages/FFT_Stage9 ==
  enable : Inport
  data_in : Inport  Port=2
  index_in : Inport  Port=3
  Butterfly_FFT2_Computing_Unit : MATLAB Function  TreatAsAtomicUnit=on
  Control_Logic : MATLAB Function  TreatAsAtomicUnit=on
  Dual Port RAM : hdlsllib/HDL RAMs/Simple Dual Port RAM  ram_size=9
  Twiddle_ROM : MATLAB Function  TreatAsAtomicUnit=on
  delay_data_en : UnitDelay
  delay_data_out : UnitDelay
  delay_index_out : Delay  DelayLength=6
  delay_index_out1 : UnitDelay
  reg_twiddle : Delay  DelayLength=3
  reg_twiddle1 : Delay
  reg_u1 : Delay
  reg_v1 : Delay  DelayLength=1
  reg_x : Delay
  reg_y : Delay
  data_en : Outport
  data_out : Outport  Port=2
  index_out : Outport  Port=3
  wires:
  Control_Logic/7(mem_wr_din) -> Dual Port RAM/1
  Control_Logic/6(index_out) -> delay_index_out/1
  Control_Logic/5(data_out) -> delay_data_out/1
  Control_Logic/4(data_en) -> delay_data_en/1
  Control_Logic/2(fft2_v) -> reg_v1/1
  reg_v1/1 -> Butterfly_FFT2_Computing_Unit/2(fft2_v)
  Dual Port RAM/1 -> Control_Logic/6(mem_rd_dout)
  reg_twiddle1/1 -> Twiddle_ROM/1(twiddle_addr)
  Twiddle_ROM/1(fft2_twiddle) -> reg_twiddle/1
  delay_index_out1/1 -> index_out/1
  delay_data_out/1 -> data_out/1
  delay_data_en/1 -> data_en/1
  index_in/1 -> Control_Logic/5(index_in)
  data_in/1 -> Control_Logic/4(data_in)
  enable/1 -> Control_Logic/3(enable)
  reg_y/1 -> Control_Logic/2(fft2_y)
  reg_x/1 -> Control_Logic/1(fft2_x)
  reg_twiddle/1 -> Butterfly_FFT2_Computing_Unit/3(fft2_twiddle)
  Control_Logic/3(twiddle_addr) -> reg_twiddle1/1
  reg_u1/1 -> Butterfly_FFT2_Computing_Unit/1(fft2_u)
  delay_index_out/1 -> delay_index_out1/1
  Butterfly_FFT2_Computing_Unit/2(fft2_y) -> reg_y/1
  Butterfly_FFT2_Computing_Unit/1(fft2_x) -> reg_x/1
  Control_Logic/1(fft2_u) -> reg_u1/1
  Control_Logic/10(mem_rd_addr) -> Dual Port RAM/4
  Control_Logic/9(mem_wr_en) -> Dual Port RAM/3
  Control_Logic/8(mem_wr_addr) -> Dual Port RAM/2

== matlab function hdlcoder_ofdm_fft_eml/FFT_512Pt_EML_Serial/Serialized_FFT/FFT_Stages/FFT_Stage3/Butterfly_FFT2_Computing_Unit ==
  settings: fimath=hdlfimath
  data: fft2_u input FFT_nt; fft2_x output FFT_nt; fft2_v input FFT_nt; fft2_twiddle input twiddle_nt; fft2_y output FFT_nt
function [fft2_x, fft2_y] = fcn(fft2_u, fft2_v, fft2_twiddle)
% FFT2 Computing Unit

% Scale down number for this stage. Need to be power of 2.
Scale = 1;

% Call function in hdlcoder_serial_fft_butterfly_scale.m on path 
[x, y] = hdlcoder_serial_fft_butterfly(fft2_u, fft2_v, fft2_twiddle);

% scaling down by 2 for each FFT2 stage.
fft2_x = bitsra(x, log2(Scale));
fft2_y = bitsra(y, log2(Scale));

== matlab function hdlcoder_ofdm_fft_eml/FFT_512Pt_EML_Serial/Serialized_FFT/FFT_Stages/FFT_Stage3/Control_Logic ==
  settings: fimath=hdlfimath
  data: fft2_x input FFT_nt; fft2_y input FFT_nt; fft2_u output FFT_nt; fft2_v output FFT_nt; twiddle_addr output; enable input boolean; data_in input FFT_nt; index_in input fixdt(0,TotalStage+1,0); data_en output boolean; data_out output FFT_nt; index_out output; mem_rd_dout input FFT_nt; mem_wr_din output FFT_nt; mem_wr_addr output; mem_wr_en output; mem_rd_addr output; TotalStage parameter
function [fft2_u, fft2_v, twiddle_addr, data_en, data_out, index_out, mem_wr_din, mem_wr_addr, mem_wr_en, mem_rd_addr] ...
          = fcn(fft2_x, fft2_y, enable, data_in, index_in, mem_rd_dout, TotalStage)
% FF2 Stages in Serial FFT Model
% Each stage is composed of one FFT2 butterfly computing unit, 
% some memory to cache the streaming data and twiddles, and some control logics.
%
% The incoming streaming data are first stored into cache memory in the data order of last stage,
% and then they are read out in the data order of current stage and send to FFT computing unit.
% The computing unit will produce one result data every clock cycle, and the data_out will streaming
% out the result data in the order of current stage.
% 
% The memory size of each stage is the same as Stage Number, except Stage 1 (the minimum size of
% the memory block is 2). So all the stages share the same code except Stage 1.
% 
% To expand the size of FFT model, user can simply copy and paste new stage blocks and insert them
% before the End_Stage_Reorder block. Only the "Stage" in this code needs to be modified in the new block. 
% And also the size of memory blocks needs to be modified in the new block.
      
Stage = 3;      

N = uint16(2^(Stage-1));
nt = numerictype(data_in);
fm = fimath(data_in);

nt1 = numerictype(0, Stage+1, 0);
nt2 = numerictype(0, Stage-1, 0);
nt3 = numerictype(0, TotalStage-Stage+1, 0);
nt_addr = numerictype(0, TotalStage+1, 0);

% State machine registers
persistent main_state butterfly_state 
nts = numerictype(0, 2, 0);
if isempty(main_state)
    main_state = getfi(0, nts);
end
if isempty(butterfly_state)
    butterfly_state = getfi(0, nts);
end

% Address counters
persistent mem_addr mem_addr1 mem_addr2 
if isempty(mem_addr)
    mem_addr  = getfi(0, nt_addr);
end
if isempty(mem_addr1)
    mem_addr1 = getfi(0, nt_addr);
end
if isempty(mem_addr2)
    mem_addr2 = getfi(0, nt_addr);
end

persistent ctr ctr_lsb1c ctr_lsb2c ctr_msb
if isempty(ctr)
    ctr       = getfi(0, nt1);
end
if isempty(ctr_lsb1c)
    ctr_lsb1c = getfi(0, nt2);
end
if isempty(ctr_lsb2c)
    ctr_lsb2c = getfi(0, nt2);
end
if isempty(ctr_msb)
    ctr_msb   = getfi(0, nt3);
end

% Input/Output
mem_rd_addr  = bitsliceget(mem_addr, Stage, 1);
mem_wr_addr  = bitsliceget(index_in, Stage, 1);
mem_wr_din   = data_in;
index_out    = mem_addr;
twiddle_addr = ctr_lsb1c;

% Delay register inserted before the FFT2 computing unit
persistent reg_u reg_v
if isempty(reg_u)
    reg_u = complex(getfi(0, nt));
end
if isempty(reg_v)
    reg_v = complex(getfi(0, nt));
end
fft2_u = reg_u;
fft2_v = reg_v;

% Main state machine control the memory and data enable signals
switch uint8(main_state)
    case 0 %initial
        mem_wr_en    = false;
        calcu_en     = false;
        data_en      = false;
        ctr_en       = false;
        if enable
            main_state = getfi(1, nts);
        else
            main_state = getfi(0, nts);
        end
        
    case 1 %write data
        mem_wr_en    = true;
        calcu_en     = false;
        data_en      = false;
        ctr_en       = true;
        if ctr == getfi(N-2, nt1)
            main_state = getfi(2, nts);
        else
            main_state = getfi(1, nts);
        end
       
    case 2 %read & calculate data
        mem_wr_en    = true;
        calcu_en     = true;
        data_en      = false;
        ctr_en       = true;
        if ctr == getfi(N+4, nt1)
            main_state = getfi(3, nts);
        else
            main_state = getfi(2, nts);
        end

    case 3 %set output data_en signal, keep calculation
        mem_wr_en    = true;
        calcu_en     = true;
        data_en      = true;
        ctr_en       = false;
        main_state   = getfi(3, nts);
        
    otherwise
        mem_wr_en    = false;
        calcu_en     = false;
        data_en      = false;
        ctr_en       = false;
        main_state   = getfi(0, nts);
end

% Butterfly calculation state machine controls the memory access and data movement
switch uint8(butterfly_state)
    case 0 %initial
        data_out    = fft2_x;
        mem_addr    = mem_addr1;
        ctr_lsb1_en = false;
        ctr_lsb2_en = false;        
        if calcu_en
            butterfly_state = getfi(1, nts);
        else
            butterfly_state = getfi(0, nts);
        end
        
    case 1 %pre-read data
        data_out    = fft2_y;    
        mem_addr    = mem_addr2;
        ctr_lsb1_en = true;
        ctr_lsb2_en = false;
        butterfly_state = getfi(2, nts);

    case 2 %read data -> reg_u
        reg_u       = mem_rd_dout;
        data_out    = fft2_y;
        mem_addr    = mem_addr1;
        ctr_lsb1_en = false;
        ctr_lsb2_en = true;
        butterfly_state = getfi(3, nts);

    case 3 %read data -> reg_v
        reg_v       = mem_rd_dout;       
        data_out    = fft2_x;
        mem_addr    = mem_addr2;
        ctr_lsb1_en = true;
        ctr_lsb2_en = false;
        butterfly_state = getfi(2, nts);   
        
    otherwise
        data_out    = fft2_y;
        mem_addr    = mem_addr1;
        ctr_lsb1_en = false;
        ctr_lsb2_en = false;
        butterfly_state = getfi(0, nts);
end

% Memory address msb counter enable signal
if (ctr_lsb1_en == true) && (ctr_lsb1c == getfi(N-1, nt2))
    ctr_msb_en = true;
else
    ctr_msb_en = false;
end

% Mem_count counter
ctr = update_counter(ctr_en, ctr, nt1);

% Memory address lsb counter 1 
ctr_lsb1c = update_counter(ctr_lsb1_en, ctr_lsb1c, nt2);

% Memory address lsb counter 2
ctr_lsb2c = update_counter(ctr_lsb2_en, ctr_lsb2c, nt2);

% Memory address msb counter
ctr_msb = update_counter(ctr_msb_en, ctr_msb, nt3);

% The output address representation
c0_ufix1 = fi(0, 0, 1, 0, fm);
c1_ufix1 = fi(1, 0, 1, 0, fm);
ctr_lsb1 = bitconcat(c0_ufix1, ctr_lsb1c);
ctr_lsb2 = bitconcat(c1_ufix1, ctr_lsb2c);
mem_addr1 = bitconcat(ctr_msb, ctr_lsb1);
mem_addr2 = bitconcat(ctr_msb, ctr_lsb2);
                  
end

function out = update_counter(enable, in, nt)
if enable
    out = getfi(in + getfi(1, nt), nt);
else
    out = in;
end
end

function f = getfi(u, nt)
f = fi(u, nt, hdlfimath);
end

== matlab function hdlcoder_ofdm_fft_eml/FFT_512Pt_EML_Serial/Serialized_FFT/FFT_Stages/FFT_Stage3/Twiddle_ROM ==
  settings: fimath=hdlfimath
  data: twiddle_addr input; fft2_twiddle output twiddle_nt; TotalPoint parameter; twiddle_Signed parameter; twiddle_WordLength parameter; twiddle_FractionLength parameter
function fft2_twiddle = fcn(twiddle_addr, TotalPoint, twiddle_Signed, twiddle_WordLength, twiddle_FractionLength)
% Twiddle ROM

Stage = 3;

nt = numerictype(twiddle_Signed, twiddle_WordLength, twiddle_FractionLength);
fm = fimath(...
'RoundMode', 'nearest',...
'OverflowMode', 'saturate',...
'ProductMode', 'FullPrecision', 'ProductWordLength', 128,...
'SumMode', 'FullPrecision', 'SumWordLength', 128,...
'CastBeforeSum', true);

% Provide twiddle data for FFT calculation
persistent twiddleValue
if isempty(twiddleValue)
    twiddleValue = fi(exp(-2*pi*1i*(0:(TotalPoint/(2^Stage)):(TotalPoint/2-1))/TotalPoint).', nt, fm);   
end
fft2_twiddle = twiddleValue(int32(twiddle_addr)+1);

== matlab function hdlcoder_ofdm_fft_eml/FFT_512Pt_EML_Serial/Serialized_FFT/FFT_Stages/FFT_Stage4/Butterfly_FFT2_Computing_Unit ==
  settings: fimath=hdlfimath
  data: fft2_u input FFT_nt; fft2_x output FFT_nt; fft2_v input FFT_nt; fft2_twiddle input twiddle_nt; fft2_y output FFT_nt
function [fft2_x, fft2_y] = fcn(fft2_u, fft2_v, fft2_twiddle)
% FFT2 Computing Unit

% Scale down number for this stage. Need to be power of 2.
Scale = 1;

% Call function in hdlcoder_serial_fft_butterfly_scale.m on path 
[x, y] = hdlcoder_serial_fft_butterfly(fft2_u, fft2_v, fft2_twiddle);

% scaling down by 2 for each FFT2 stage.
fft2_x = bitsra(x, log2(Scale));
fft2_y = bitsra(y, log2(Scale));
